simulink model "FMS"  (R2018b)
settings: configuration reference "fms_config" (kept outside this file)
values from neighbouring files (symbols this model uses):
  FMS_EXPORT = Simulink.Parameter(FMS_EXPORT_VALUE)    [fms_model_init.m]
  FMS_PARAM = Simulink.Parameter(FMS_PARAM_VALUE)    [fms_model_init.m]
undefined symbols (not defined in the file or in its folder): actuator_cmd, ax_cmd, ay_cmd, az_cmd, cmd_mask, ControlMode, ctrl_mode, DiscIntNeverNeededParam, FMS_Cmd, FMS_CONST, FMS_Error, home, mode, p_cmd, phi_cmd, PilotMode, psi_rate_cmd, q_cmd, r_cmd, reset, state, status, theta_cmd, throttle_cmd, timestamp, u_cmd, v_cmd, VehicleState, VehicleStatus, w_cmd, wp_consume, wp_current
libraries: simulink x123, FMT_Model_Lib x62, hdlsllib x13
(part 7 of 7)

== stateflow chart FMS/FMS Commander/Commander/Arm/Assist/Position/Altitude Command/Detect Movement/Motion Status ==
  state Hold
    entry:
    state=MotionState.Hold;
  state Move
    entry:
    state=MotionState.Move;
  state Brake
    entry:
    state=MotionState.Brake;
  (default) -> Move
  Hold -> Move : [motion_req==1]
  Move -> Brake : [motion_req==0]
  Brake -> Move [order 2] : [motion_req==1]
  Brake -> Hold [order 1] : [speed<=0.15 || after(1.5, sec)]
  data: state output Enum: MotionState; motion_req input; speed input

== stateflow chart FMS/FMS Commander/Commander/Arm/Auto/Mission/Mission_SubSystem/Velocity Commander/Hold Position/Altitude Hold/Detect Movement/Motion Status ==
  state Hold
    entry:
    state=MotionState.Hold;
  state Move
    entry:
    state=MotionState.Move;
  state Brake
    entry:
    state=MotionState.Brake;
  (default) -> Move
  Hold -> Move : [motion_req==1]
  Move -> Brake : [motion_req==0]
  Brake -> Move [order 2] : [motion_req==1]
  Brake -> Hold [order 1] : [speed<=0.15 || after(1.5, sec)]
  data: state output Enum: MotionState; motion_req input; speed input

== stateflow chart FMS/FMS Commander/Commander/Arm/Auto/Mission/Mission_SubSystem/Velocity Commander/Hold Position/Position Hold/Detect Movement/Motion State ==
  state Hold
    entry:
    state=MotionState.Hold;
  state Move
    entry:
    state=MotionState.Move;
  state Brake
    entry:
    state=MotionState.Brake;
  (default) -> Move
  Hold -> Move : [motion_req==1]
  Move -> Brake : [motion_req==0]
  Brake -> Move [order 2] : [motion_req==1]
  Brake -> Hold [order 1] : [speed<=0.2 || after(2.5, sec)]
  data: state output Enum: MotionState; motion_req input; speed input

== matlab function FMS/FMS Commander/Commander/Arm/Auto/Mission/Mission_SubSystem/Velocity Commander/L1 Reference WP/NearbyRefWP ==
  data: P output; P2 input; d output; P3 input; L1 input
% Find the reference waypoint when vehicle (P3) is close to target (P2)
%
% If the vehicle is close to target (distance(P2,P3) < L1), select P2 as
% reference waypoint and return the distance, otherwise return -1.
function [P,d] = NearbyRefWP(P2, P3, L1)

P3P2 = P2 - P3;
dis = sqrt(sum(P3P2.^2));

if dis <= L1
    d = dis;
    % select P2 as reference WP
    P = P2;
else
    d = single(-1);
    % unset WP
    P = single([0; 0]);
end

== stateflow chart FMS/FMS Commander/Commander/Arm/Assist/Position/Heading Command/Detect Movement/Motion State ==
  state Hold
    entry:
    state=MotionState.Hold;
  state Move
    entry:
    state=MotionState.Move;
  state Brake
    entry:
    state=MotionState.Brake;
  (default) -> Move
  Hold -> Move : [motion_req==1]
  Move -> Brake : [motion_req==0]
  Brake -> Move [order 2] : [motion_req==1]
  Brake -> Hold [order 1] : [speed<=0.1 || after(1, sec)]
  data: state output Enum: MotionState; motion_req input; speed input

== matlab function FMS/FMS Commander/Commander/Arm/Auto/Mission/Mission_SubSystem/Velocity Commander/L1 Reference WP/OutRegionRegWP ==
  data: P1 input; P output; P2 input; P3 input
% Find the reference waypoint when vehicle is out of L1 region near P1P2.
%
% There are three region defined:
%   Region 1: The project point of P3 is lied on left side of P1P2
%   Region 2: The project point of P3 is lied on right side of P1P2
%   Region 3: The project point of P3 is lied on the segment line 
%
%   For the case of region 3, we select the project point as the reference
%   wayspoint. For the case of region 1, we choose P1 as reference waypoint
%   and similarly for the case of region 2, we choose P3 as reference
%   waypoint.
function P = OutRegionRefWP(P1, P2, P3)
% segment line P1P2
P1P2 = P2 - P1;
% segment line P1P3
P1P3 = P3 - P1;

% Define C as the P3 project point on line P1P2.
% Hence, P1C = dot(P1P3, P1P2)/|P1P2| * (P1P2/|P1P2|) = u * P1P2
% where u = dot(P1P3, P1P2) / |P1P2|^2.
u = dot(P1P3, P1P2) / sum(P1P2.^2);

if u <= 0
    % region 1
    P = P1;
elseif u >= 1
    % region 2
    P = P2;
else
    % region 3. C = P1C + P1
    P = u * P1P2 + P1;
end

== matlab function FMS/FMS Commander/Commander/Arm/Auto/Mission/Mission_SubSystem/Velocity Commander/L1 Reference WP/SearchL1RefWP ==
  data: P1 input; P output; P2 input; P3 input; L1 input; u output
% Find reference waypoint (L1RefWP) on the line segment P1P2 which has 
% L1 distance from vehicle position (P3).
%
% The idea is to calculate the intersection point of a circle with L1 radius
% with the line segment P1P2.
%
% Define P = P1 + u * (P2 - P1), where P is the intersection point.
% Goal is calculating the u, where the valid u is between [0, 1].
%
% Input:
%   P1: start point of segment line
%   P2: start point of segment line
%   P3: circle center point, also is known as the vehicle position
%   L1: the L1 distance
% Output:
%   P: L1 reference waypoint
%   u: scale factor (valid between 0 and 1), -1 means no intersection.
function [P, u] = SearchL1RefWP(P1, P2, P3, L1)

% P1 = (x1, y1), P2 = (x2, y2), P3 = (x3, y3)
x1 = P1(1);
y1 = P1(2);
x2 = P2(1);
y2 = P2(2);
x3 = P3(1);
y3 = P3(2);

% The P is on circle and line segment, which yields:
A = (x2 - x1)^2 + (y2 - y1)^2;
B = 2 * ((x2 - x1)*(x1 - x3) + (y2 - y1)*(y1 - y3));
C = x3^2 + y3^2 + x1^2 + y1^2 - 2*(x3*x1 + y3*y1) - L1^2;
% Check root existence confition if B^2 - 4*A*C >= 0
D = B^2 - 4*A*C;
u = single(-1);
P = single([0 0]);

if D > 0
    % D>0 means we have 2 difference roots, % root is valid only if u is in range of [0, 1]
    u1 = (-B + sqrt(D)) / (2*A);
    u2 = (-B - sqrt(D)) / (2*A);
    
    if (u1>=0 && u1<=1) && (u2>=0 && u2<=1)
        % have 2 valid roots, select the one which is closer to P2 (target point)
        if u1 > u2
            u = u1; 
        else
            u = u2;
        end
    elseif (u1>=0 && u1<=1)
        % only 1 root valid, select it
        u = u1;
    elseif (u2>=0 && u2<=1)
        % only 1 root valid, select it
        u = u2;
    else
        % no valid root, which means no intersection point founded.
        return;
    end
elseif D == 0
    % D=0 means only 1 single root
    u1 = -B / (2*A);
    if (u1>=0 && u1<=1)
        % valid root, select it
        u = u1;
    else
        % no valid root, which means no intersection point founded.
        return;
    end
else
    % no valid root, which means no intersection point founded.
    return;
end

% calculate the L1 reference waypoint (P) coordinate
P(1) = x1 + u*(x2 - x1);
P(2) = y1 + u*(y2 - y1);

== stateflow chart FMS/FMS Commander/Commander/Arm/SubMode/Return/Velocity Commander/Hold Position/Altitude Hold/Detect Movement/Motion Status ==
  state Hold
    entry:
    state=MotionState.Hold;
  state Move
    entry:
    state=MotionState.Move;
  state Brake
    entry:
    state=MotionState.Brake;
  (default) -> Move
  Hold -> Move : [motion_req==1]
  Move -> Brake : [motion_req==0]
  Brake -> Move [order 2] : [motion_req==1]
  Brake -> Hold [order 1] : [speed<=0.15 || after(1.5, sec)]
  data: state output Enum: MotionState; motion_req input; speed input

== stateflow chart FMS/FMS State Machine ==
  state Command_Listener [parallel]
    settings: executionOrder=1
    state Send
      entry:
      % Send command
      M.data=save_cmd;
      send(M);
    state Listen
    state Check
      entry:
      valid_cmd = CheckCmdValid(save_cmd, mode, INS_Out.flag, fms_error);
    (default) -> Listen
    Send -> Listen
    Check -> Listen [order 2]
    Listen -> Check : [hasChanged(cmd) && ...
        | cmd ~= FMS_Cmd.None]{save_cmd = cmd;}
    Check -> Send [order 1] : [valid_cmd == true]
  state Vehicle [parallel]
    du:
    % if mission data updated, reset waypoint index
    if hasChanged(mission_timestamp)
    wp_consume = 0;
    wp_index = 1;
    end
    settings: executionOrder=4
    state moved = StickMoved(stick_val,pilot_cmd) [function]
    state sp_takeoff = PrepTakeoff(xy_R) [function]
    state Arm
      en:
      status = VehicleStatus.Arm;
      state SubMode
        en:
        % save enter stick value
        stick_val = [Pilot_Cmd.stick_yaw; Pilot_Cmd.stick_throttle; Pilot_Cmd.stick_roll; Pilot_Cmd.stick_pitch];
        state Return
          en:
          state = VehicleState.Return;
        state Land
          en:
          state = VehicleState.Land;
        state Takeoff
          en:
          state = VehicleState.Takeoff;
        state Hold
          en:
          state = VehicleState.Hold;
        Vehicle.Arm.SubMode.Return -> Vehicle.Arm.SubMode.Land : [norm([INS_Out.x_R,INS_Out.y_R]-[home(1),home(2)]) ...
            | <= accept_radius]
            | {Cmd_In.sp_waypoint = [home(1); home(2); 0]}
        Vehicle.Arm.SubMode.Takeoff -> (junction 612) : [INS_Out.h_R >= Cmd_In.sp_waypoint(3)]
        (junction 612) -> Vehicle.Arm.SubMode.Hold [order 2]
      state Auto
        state Offboard
          state Loiter
            en:
            state = VehicleState.Hold;
          state Run
            en:
            state = VehicleState.Offboard;
          (default) -> (junction 958)
          (junction 958) -> Vehicle.Arm.Auto.Offboard.Loiter [order 2]
          (junction 958) -> Run [order 1] : [auto_cmd_valid == 1]
          Run -> Vehicle.Arm.Auto.Offboard.Loiter : [auto_cmd_valid == 0]
          Vehicle.Arm.Auto.Offboard.Loiter -> Run : [auto_cmd_valid == 1]
        state Mission
          en:
          % Reference location of latitude and longitude, specified as an m-by-2 array, in degrees
          llo = [INS_Out.lat_0, INS_Out.lon_0] * (180/pi);
          % Set setpoint waypoint to current position
          Cmd_In.sp_waypoint = [INS_Out.x_R; INS_Out.y_R; INS_Out.h_R];
          % Init set_speed and set_yaw
          Cmd_In.set_speed = single(0);
          Cmd_In.set_yaw = single(-1);
          state pos = LLA2FLAT(lla,llo,href,psio) [function]
          state Takeoff_Waypoint
            en:
            % Geodetic coordinates (latitude, longitude, and altitude), specified as an m-by-3 array in [degrees degrees meters]
            % Altitude add home(3) here because the altitude when takeoff could be non-zero
            lla = [double(Mission_Data.x(wp_index))*1e-7, double(Mission_Data.y(wp_index))*1e-7, double(-(Mission_Data.z(wp_index) + home(3)))];
            % set takeoff setpoint
            Cmd_In.cur_waypoint = [INS_Out.x_R; INS_Out.y_R; INS_Out.h_R];
            Cmd_In.sp_waypoint = LLA2FLAT(lla, llo, 0, 0);
            % enter mission state
            state = VehicleState.Mission;
          state Loiter
            en:
            state = VehicleState.Hold;
          state NextWP
            en:
            if wp_index <= Mission_Data.valid_items
            nav_cmd = Mission_Data.command(wp_index);
            else
            nav_cmd = uint16(NAV_Cmd.None);
            % updated consumed waypoints
            wp_consume = wp_index - 1;
            end
          state Takeoff
            en:
            % Geodetic coordinates (latitude, longitude, and altitude), specified as an m-by-3 array in [degrees degrees meters]
            % Altitude add home(3) here because the altitude when takeoff could be non-zero
            lla = [double(Mission_Data.x(wp_index))*1e-7, double(Mission_Data.y(wp_index))*1e-7, double(-(Mission_Data.z(wp_index) + home(3)))];
            % set takeoff setpoint
            Cmd_In.cur_waypoint = [INS_Out.x_R; INS_Out.y_R; INS_Out.h_R];
            Cmd_In.sp_waypoint = LLA2FLAT(lla, llo, 0, 0);
            Cmd_In.sp_waypoint(1:2) = reachable_wp(Cmd_In.cur_waypoint, Cmd_In.sp_waypoint);
            % enter takeoff state
            state = VehicleState.Takeoff;
            state reachable_wp = reachable_wp(cur_waypoint,sp_waypoint) [function]
          state Waypoint
            en:
            % Geodetic coordinates (latitude, longitude, and altitude), specified as an m-by-3 array in [degrees degrees meters]
            % Altitude add home(3) here because the altitude when takeoff could be non-zero
            lla = [double(Mission_Data.x(wp_index))*1e-7, double(Mission_Data.y(wp_index))*1e-7, double(-(Mission_Data.z(wp_index) + home(3)))];
            % set current waypoint to previous setpoint waypoint
            Cmd_In.cur_waypoint = Cmd_In.sp_waypoint;
            % target waypoint
            Cmd_In.sp_waypoint = LLA2FLAT(lla, llo, 0, 0);
            % set yaw
            if Mission_Data.param4(wp_index) >= 0
            Cmd_In.set_yaw = Mission_Data.param4(wp_index)/180*pi;
            else
            Cmd_In.set_yaw = atan2(Cmd_In.sp_waypoint(2)-Cmd_In.cur_waypoint(2), Cmd_In.sp_waypoint(1)-Cmd_In.cur_waypoint(1));
            end
            state = VehicleState.Mission;
          state Disarming
          state Hold
            en:
            state = VehicleState.Hold;
          state SetSpeed
            en:
            % set cruise speed
            Cmd_In.set_speed = Mission_Data.param2(wp_index);
          state Land
            en:
            Cmd_In.sp_waypoint = [INS_Out.x_R; INS_Out.y_R; 0];
            state = VehicleState.Land;
          state Return
            en:
            Cmd_In.sp_waypoint = [home(1); home(2); INS_Out.h_R];
            state = VehicleState.Return;
          Mission -> NextWP : [hasChanged(mission_timestamp)]
          (junction 908) -> (junction 910) : {wp_index = wp_index + 1;}
          (junction 910) -> NextWP
          (junction 873) -> (junction 908)
          (default) -> NextWP
          Takeoff_Waypoint -> (junction 873) : [norm([INS_Out.x_R;INS_Out.y_R;INS_Out.h_R]-Cmd_In.sp_waypoint(1:3)) <= accept_radius]
          (junction 1010) -> Takeoff_Waypoint [order 1] : [norm([INS_Out.x_R;INS_Out.y_R]-Cmd_In.sp_waypoint(1:2)) <= accept_radius]
          NextWP -> Vehicle.Arm.Auto.Mission.Takeoff [order 1] : [nav_cmd == NAV_Cmd.Takeoff]
          Vehicle.Arm.Auto.Mission.Takeoff -> (junction 1010) : [INS_Out.h_R >= Cmd_In.sp_waypoint(3)]
          (junction 1010) -> (junction 873) [order 2]
          (junction 917) -> Vehicle.Arm.Auto.Mission.Loiter [order 2]
          (junction 879) -> (junction 873)
          NextWP -> (junction 917) [order 6]
          (junction 917) -> Disarming [order 1] : [on_ground]
          NextWP -> Waypoint [order 2] : [nav_cmd == NAV_Cmd.Waypoint]
          Waypoint -> (junction 997) : [norm([INS_Out.x_R;INS_Out.y_R;INS_Out.h_R]-Cmd_In.sp_waypoint(1:3)) <= accept_radius]
              | {Cmd_In.set_speed = single(0); Cmd_In.set_yaw = single(-1);}
          (junction 997) -> (junction 879) [order 2]
          (junction 997) -> Vehicle.Arm.Auto.Mission.Hold [order 1] : [Mission_Data.param1(wp_index) > 0]
          Vehicle.Arm.Auto.Mission.Hold -> (junction 879) : after(Mission_Data.param1(wp_index),sec)
          (junction 994) -> (junction 879)
          NextWP -> SetSpeed [order 3] : [nav_cmd == NAV_Cmd.SetSpeed]
          SetSpeed -> (junction 994)
          (junction 915) -> (junction 994)
          NextWP -> Vehicle.Arm.Auto.Mission.Return [order 5] : [nav_cmd == NAV_Cmd.Return]
          NextWP -> Vehicle.Arm.Auto.Mission.Land [order 4] : [nav_cmd == NAV_Cmd.Land]
          Vehicle.Arm.Auto.Mission.Land -> (junction 915) : [duration(on_ground) >= 2]
          Vehicle.Arm.Auto.Mission.Return -> Vehicle.Arm.Auto.Mission.Land : [norm([INS_Out.x_R; INS_Out.y_R]-Cmd_In.sp_waypoint(1:2)) < 0.5]
        state InvalidAutoMode
        (default) -> (junction 43)
        (junction 43) -> Offboard [order 1] : [mode == PilotMode.Offboard]
        (junction 43) -> (junction 134) [order 2]
        (junction 134) -> Mission [order 1] : [mode == PilotMode.Mission]
        (junction 134) -> InvalidAutoMode [order 2]
        Disarming -> (junction 370)
        InvalidAutoMode -> (junction 370)
      state Assist
        state InvalidAssistMode
        state Acro
          en:
          state = VehicleState.Acro;
        state Stabilize
          en:
          state = VehicleState.Stabilize;
        state Altitude
          en:
          state = VehicleState.Altitude;
        state Position
          en:
          state = VehicleState.Position;
        (default) -> (junction 354)
        (junction 354) -> (junction 190) [order 2]
        (junction 190) -> (junction 193) [order 2]
        (junction 193) -> (junction 196) [order 2]
        (junction 196) -> InvalidAssistMode [order 2]
        (junction 354) -> Acro [order 1] : [mode == PilotMode.Acro]
        (junction 190) -> Stabilize [order 1] : [mode == PilotMode.Stabilize]
        (junction 193) -> Altitude [order 1] : [mode == PilotMode.Altitude]
        (junction 196) -> Position [order 1] : [mode == PilotMode.Position]
      state Manual
        state InValidManualMode
        state Manual
          en:
          state = VehicleState.Manual;
        (default) -> (junction 410)
        (junction 410) -> InValidManualMode [order 2]
        (junction 410) -> Vehicle.Arm.Manual.Manual [order 1] : [mode == PilotMode.Manual]
      state InvalidArmMode
      Vehicle.Arm -> Vehicle.Arm.SubMode.Land [order 3] : M[M.data==FMS_Cmd.Land]
          | {Cmd_In.sp_waypoint = [INS_Out.x_R; INS_Out.y_R; 0]}
      Vehicle.Arm -> Vehicle.Arm.SubMode.Hold [order 1] : M[M.data==FMS_Cmd.Pause]
      Vehicle.Arm -> Vehicle.Arm.SubMode.Return [order 4] : M[M.data==FMS_Cmd.Return]
          | {Cmd_In.cur_waypoint = [INS_Out.x_R; INS_Out.y_R; INS_Out.h_R];
          | Cmd_In.sp_waypoint = [home(1); home(2); INS_Out.h_R]}
      Vehicle.Arm.SubMode.Hold -> Vehicle.Arm : M[M.data==FMS_Cmd.Continue ...
          | && mode ~= PilotMode.None]
      (junction 612) -> (junction 117) [order 1] : [mode ~= PilotMode.None]
      SubMode -> (junction 117) : [(StickMoved(stick_val, Pilot_Cmd) || ...
          | bitand(INS_Out.flag, 212) ~= 212) && ...
          | mode ~= PilotMode.None]
      Vehicle.Arm -> (junction 117) [order 2] : [hasChanged(mode) && ...
          | mode ~= PilotMode.None]
      (junction 117) -> Auto [order 1] : [getArmMode(mode) == 3]
      (default) -> (junction 117)
      (junction 117) -> (junction 140) [order 2]
      (junction 140) -> Assist [order 1] : [getArmMode(mode)  == 2]
      (junction 140) -> (junction 240) [order 2]
      (junction 240) -> Vehicle.Arm.Manual [order 1] : [getArmMode(mode)  == 1]
      (junction 240) -> InvalidArmMode [order 2]
    state Standby
      en:
      % check if mission takeoff is valid
      if mode==PilotMode.Mission
      if (wp_index <= Mission_Data.valid_items && ...
      Mission_Data.command(wp_index)==NAV_Cmd.Takeoff) || ...
      (wp_index+1 <= Mission_Data.valid_items && ...
      Mission_Data.command(wp_index)==NAV_Cmd.SetSpeed && ...
      Mission_Data.command(wp_index+1)==NAV_Cmd.Takeoff)
      % set mission takeoff flag, so enter mission mode after 2s
      prep_mission_takeoff = 1;
      % unset prep_takeoff if prep_mission_takeoff=1
      prep_takeoff = 0;
      else
      send(DisarmEvent);
      end
      end
      % set current position as home
      home = [INS_Out.x_R; INS_Out.y_R; INS_Out.h_R; INS_Out.psi];
      % enter standby state
      state = VehicleState.Standby;
      status = VehicleStatus.Standby;
      ex:
      % on exit, unset takeoff flag
      prep_takeoff = 0;
      prep_mission_takeoff = 0;
    state Disarm
      en:
      state = VehicleState.Disarm;
      status = VehicleStatus.Disarm;
    InValidManualMode -> Vehicle
    Vehicle.Arm.SubMode.Land -> (junction 330) : [duration(on_ground) >= 2]
    (junction 330) -> Vehicle.Disarm
    (junction 332) -> (junction 334)
    (junction 334) -> Vehicle.Arm.SubMode.Takeoff : {Cmd_In.cur_waypoint = [INS_Out.x_R; INS_Out.y_R; INS_Out.h_R];
        | Cmd_In.sp_waypoint = PrepTakeoff([INS_Out.x_R; INS_Out.y_R]);
        | Cmd_In.sp_waypoint(3) = Cmd_In.sp_waypoint(3) + home(3);}
    Standby -> (junction 332) [order 2] : M[M.data==FMS_Cmd.Takeoff]
    Standby -> (junction 334) [order 1] : [duration(prep_takeoff == 1) >= 2]
    (junction 989) -> Vehicle.Arm.SubMode.Hold
    (junction 987) -> (junction 989) : [pilot_cmd_lost && bitand(INS_Out.flag, 212) == 212]
    InvalidAssistMode -> Vehicle
    (junction 370) -> Vehicle
    (default) -> Vehicle.Disarm
    Assist -> (junction 987)
    Standby -> Vehicle.Disarm [order 3] : after(10, sec) || DisarmEvent
    Vehicle.Disarm -> Standby [order 1] : M[M.data==FMS_Cmd.PreArm]
    Standby -> Vehicle.Arm [order 6] : [ManualArmEvent(Pilot_Cmd) == 1 &&...
        | mode ~= PilotMode.None &&...
        | prep_takeoff ~= 1]
    Vehicle.Disarm -> Standby [order 2] : M[M.data==FMS_Cmd.Takeoff]
        | {prep_takeoff = 1;}
    Standby -> Vehicle.Arm [order 5] : [mode == PilotMode.Offboard && ...
        | auto_cmd_valid && prep_takeoff ~= 1]
    Vehicle -> Vehicle.Disarm : M[M.data==FMS_Cmd.Disarm]
    (junction 304) -> Vehicle.Disarm
    Standby -> (junction 903) [order 4] : [duration(prep_mission_takeoff == 1) >= 2]
    (junction 903) -> Vehicle.Arm
    Vehicle.Arm -> (junction 304) [order 1] : [duration(on_ground) >= 2 && mode ~= PilotMode.Mission]
    InvalidArmMode -> Vehicle
  state Combo_Stick [parallel]
    settings: executionOrder=2
    state res = BottomRight(pilot_cmd) [function]
      (default) -> (junction 285) : {res = (pilot_cmd.stick_throttle < -0.8) && ...
          | (pilot_cmd.stick_yaw > 0.8);}
    state Idle
      du:
      bl = BottomLeft(Pilot_Cmd);
      br = BottomRight(Pilot_Cmd);
    state Arm
      en:
      M.data=FMS_Cmd.PreArm;
      send(M);
    state res = BottomLeft(pilot_cmd) [function]
      (default) -> (junction 298) : {res = (pilot_cmd.stick_throttle < -0.8) && ...
          | (pilot_cmd.stick_yaw < -0.8);}
    state Disarm
      en:
      send(DisarmEvent, Vehicle)
    (default) -> Idle
    Combo_Stick.Arm -> Idle : [~BottomRight(Pilot_Cmd)]
    Idle -> Combo_Stick.Arm [order 1] : [duration(br)>1.5]
    Idle -> Combo_Stick.Disarm [order 2] : [duration(bl)>1.5]
    Combo_Stick.Disarm -> Idle : [~BottomLeft(Pilot_Cmd)]
  state Lost_Return [parallel]
    settings: executionOrder=3
    state Lost
      en:
      % check if INS valid to return
      if bitand(INS_Out.flag, 221)
      M.data=FMS_Cmd.Return;
      send(M);
      end
    state Connect
    (default) -> Connect
    Connect -> Lost : [lost_connect]
    Lost -> Connect : [~lost_connect]
  data: cmd_in function_input; mode_in function_input; valid function_output; ins_flag function_input; error function_input; pilotMode function_input; armMode function_output; pilot_cmd function_input; trigger function_output; stick_val function_input double size=4; moved function_output; pilot_cmd function_input Bus: Pilot_Cmd_Bus size=1; xy_R function_input single size=2; sp_takeoff function_output; lla function_input double size=[1 3]; llo function_input double size=[1 2]; href function_input double size=1; pos function_output; psio function_input double size=1; cur_waypoint function_input single size=3; sp_waypoint function_input single size=3; reachable_wp function_output single size=2; res function_output; pilot_cmd function_input; res function_output; pilot_cmd function_input; state output Enum: VehicleState; cmd input; valid_cmd local; M local Enum: FMS_Cmd; mode input; Pilot_Cmd input Bus: Pilot_Cmd_Bus; lost_connect input; pilot_cmd_lost input; INS_Out input Bus: INS_Out_Bus; Mission_Data input Bus: Mission_Data_Bus; prep_takeoff local =0; stick_val local; bl local =false; br local =false; nav_cmd local uint16; wp_consume output uint8 =uint8(0); wp_index output uint8 =uint8(1); Cmd_In output Bus: Commander_In_Bus; mission_timestamp input uint32 =uint32(0); on_ground input; auto_cmd_valid input; status local Enum: VehicleStatus =VehicleStatus.None; llo local; lla local; prep_mission_takeoff local =0; save_cmd local Enum: FMS_Cmd; accept_radius input; home data_store_memory; fms_error input
  events: DisarmEvent local FUNCTION_CALL_EVENT
  function valid = CheckCmdValid(cmd_in, mode_in, ins_flag, error):
    | function valid = CheckCmdValid(cmd_in, mode_in, ins_flag, error)
    | 
    | % bit1 |    bit2    |    bit3  |   bit4  | bit5  | bit6  |bit7|bit8|bit9
    | % init | standstill | attitude | heading | speed | LLA   | xy | h | h_AGL
    | 
    | valid = false;
    | 
    | % TODO: Add more checks
    | switch cmd_in
    |     case {FMS_Cmd.Takeoff, FMS_Cmd.Land, FMS_Cmd.Return, FMS_Cmd.Pause}
    |         if ~bitget(ins_flag, 1) || ~bitget(ins_flag, 3) || ~bitget(ins_flag, 4)
    |             return;
    |         end
    |         % these modes need position valid
    |         if bitget(ins_flag, 5) && bitget(ins_flag, 7) && bitget(ins_flag, 8)
    |             valid = true;
    |         end
    |         
    |         if cmd_in == FMS_Cmd.Takeoff && error ~= 0
    |            valid = false; 
    |         end
    |     case FMS_Cmd.PreArm
    |         if ~bitget(ins_flag, 1) || ~bitget(ins_flag, 3) || ~bitget(ins_flag, 4) || error ~= 0
    |             return;
    |         end
    |         
    |         switch mode_in
    |             case {PilotMode.Position, PilotMode.Mission, PilotMode.Offboard}
    |                 if bitget(ins_flag, 5) && bitget(ins_flag, 7) && bitget(ins_flag, 8)
    |                     valid = true;
    |                 end
    |             case PilotMode.Altitude
    |                 if bitget(ins_flag, 8)
    |                     valid = true;
    |                 end
    |             case PilotMode.Stabilize
    |                 valid = true;
    |             otherwise
    |                 % do nothing
    |         end
    |     case FMS_Cmd.Continue
    |         if mode_in == PilotMode.Offboard || mode_in == PilotMode.Mission
    |            valid = true; 
    |         end
    |     case FMS_Cmd.Disarm
    |         valid = true;   % always allowed disarm
    |     otherwise
    |         % do nothing
    | end
    | 
    | return;
  function armMode = getArmMode(pilotMode):
    | function armMode = getArmMode(pilotMode)
    | 
    | % Map pilot mode to arm mode
    | switch pilotMode
    |     case PilotMode.Manual
    |         armMode = 1;    % manual
    |     case {PilotMode.Acro, PilotMode.Stabilize, PilotMode.Altitude, PilotMode.Position}
    |         armMode = 2;    % asist
    |     case {PilotMode.Mission, PilotMode.Offboard}
    |         armMode = 3;    % auto
    |     otherwise
    |         armMode = 0;    % unknown
    | end
    | 
    | end
  function trigger = ManualArmEvent(pilot_cmd):
    | function trigger = ManualArmEvent(pilot_cmd)
    | 
    | trigger = 0;
    | 
    | % Map pilot mode to arm mode
    | switch pilot_cmd.mode
    |     case {PilotMode.Manual, PilotMode.Acro, PilotMode.Stabilize}
    |         if pilot_cmd.stick_throttle > -0.7
    |             trigger = 1;
    |         end
    |     case {PilotMode.Altitude, PilotMode.Position}
    |         if pilot_cmd.stick_throttle > 0.1
    |             trigger = 1;
    |         end
    |     otherwise
    |         % do nothing
    | end
    | 
    | end

== stateflow chart FMS/FMS Commander/Commander/Arm/SubMode/Hold/Altitude Hold/Detect Movement/Motion Status ==
  state Hold
    entry:
    state=MotionState.Hold;
  state Move
    entry:
    state=MotionState.Move;
  state Brake
    entry:
    state=MotionState.Brake;
  (default) -> Move
  Hold -> Move : [motion_req==1]
  Move -> Brake : [motion_req==0]
  Brake -> Move [order 2] : [motion_req==1]
  Brake -> Hold [order 1] : [speed<=0.15 || after(1.5, sec)]
  data: state output Enum: MotionState; motion_req input; speed input

== stateflow chart FMS/FMS Commander/Commander/Arm/SubMode/Hold/Heading Hold/Detect Movement/Motion State ==
  state Hold
    entry:
    state=MotionState.Hold;
  state Move
    entry:
    state=MotionState.Move;
  state Brake
    entry:
    state=MotionState.Brake;
  (default) -> Move
  Hold -> Move : [motion_req==1]
  Move -> Brake : [motion_req==0]
  Brake -> Move [order 2] : [motion_req==1]
  Brake -> Hold [order 1] : [speed<=0.1 || after(1, sec)]
  data: state output Enum: MotionState; motion_req input; speed input

== stateflow chart FMS/FMS Commander/Commander/Arm/Assist/Position/Position Command/Detect Movement/Motion State ==
  state Hold
    entry:
    state=MotionState.Hold;
  state Move
    entry:
    state=MotionState.Move;
  state Brake
    entry:
    state=MotionState.Brake;
  (default) -> Move
  Hold -> Move : [motion_req==1]
  Move -> Brake : [motion_req==0]
  Brake -> Move [order 2] : [motion_req==1]
  Brake -> Hold [order 1] : [speed<=0.25 || after(3, sec)]
  data: state output Enum: MotionState; motion_req input; speed input

== stateflow chart FMS/FMS Commander/Commander/Arm/Assist/Altitude/Altitude Command/Detect Movement/Motion Status ==
  state Hold
    entry:
    state=MotionState.Hold;
  state Move
    entry:
    state=MotionState.Move;
  state Brake
    entry:
    state=MotionState.Brake;
  (default) -> Move
  Hold -> Move : [motion_req==1]
  Move -> Brake : [motion_req==0]
  Brake -> Move [order 2] : [motion_req==1]
  Brake -> Hold [order 1] : [speed<=0.15 || after(1.5, sec)]
  data: state output Enum: MotionState; motion_req input; speed input

== stateflow chart FMS/FMS Commander/Commander/Arm/Assist/Stabilize/Heading Command/Detect Movement/Motion State ==
  state Hold
    entry:
    state=MotionState.Hold;
  state Move
    entry:
    state=MotionState.Move;
  state Brake
    entry:
    state=MotionState.Brake;
  (default) -> Move
  Hold -> Move : [motion_req==1]
  Move -> Brake : [motion_req==0]
  Brake -> Move [order 2] : [motion_req==1]
  Brake -> Hold [order 1] : [speed<=0.1 || after(1, sec)]
  data: state output Enum: MotionState; motion_req input; speed input

== stateflow chart FMS/FMS Commander/Commander/Arm/SubMode/Hold/Position Hold/Detect Movement/Motion State ==
  state Hold
    entry:
    state=MotionState.Hold;
  state Move
    entry:
    state=MotionState.Move;
  state Brake
    entry:
    state=MotionState.Brake;
  (default) -> Move
  Hold -> Move : [motion_req==1]
  Move -> Brake : [motion_req==0]
  Brake -> Move [order 2] : [motion_req==1]
  Brake -> Hold [order 1] : [speed<=0.2 || after(2.5, sec)]
  data: state output Enum: MotionState; motion_req input; speed input

== stateflow chart FMS/FMS Commander/Commander/Arm/SubMode/Return/Velocity Commander/Hold Position/Position Hold/Detect Movement/Motion State ==
  state Hold
    entry:
    state=MotionState.Hold;
  state Move
    entry:
    state=MotionState.Move;
  state Brake
    entry:
    state=MotionState.Brake;
  (default) -> Move
  Hold -> Move : [motion_req==1]
  Move -> Brake : [motion_req==0]
  Brake -> Move [order 2] : [motion_req==1]
  Brake -> Hold [order 1] : [speed<=0.2 || after(2.5, sec)]
  data: state output Enum: MotionState; motion_req input; speed input

== matlab function FMS/FMS Commander/Commander/Arm/SubMode/Return/Velocity Commander/L1 Reference WP/NearbyRefWP ==
  data: P output; P2 input; d output; P3 input; L1 input
% Find the reference waypoint when vehicle (P3) is close to target (P2)
%
% If the vehicle is close to target (distance(P2,P3) < L1), select P2 as
% reference waypoint and return the distance, otherwise return -1.
function [P,d] = NearbyRefWP(P2, P3, L1)

P3P2 = P2 - P3;
dis = sqrt(sum(P3P2.^2));

if dis <= L1
    d = dis;
    % select P2 as reference WP
    P = P2;
else
    d = single(-1);
    % unset WP
    P = single([0; 0]);
end

== matlab function FMS/FMS Commander/Commander/Arm/SubMode/Return/Velocity Commander/L1 Reference WP/OutRegionRegWP ==
  data: P1 input; P output; P2 input; P3 input
% Find the reference waypoint when vehicle is out of L1 region near P1P2.
%
% There are three region defined:
%   Region 1: The project point of P3 is lied on left side of P1P2
%   Region 2: The project point of P3 is lied on right side of P1P2
%   Region 3: The project point of P3 is lied on the segment line 
%
%   For the case of region 3, we select the project point as the reference
%   wayspoint. For the case of region 1, we choose P1 as reference waypoint
%   and similarly for the case of region 2, we choose P3 as reference
%   waypoint.
function P = OutRegionRefWP(P1, P2, P3)
% segment line P1P2
P1P2 = P2 - P1;
% segment line P1P3
P1P3 = P3 - P1;

% Define C as the P3 project point on line P1P2.
% Hence, P1C = dot(P1P3, P1P2)/|P1P2| * (P1P2/|P1P2|) = u * P1P2
% where u = dot(P1P3, P1P2) / |P1P2|^2.
u = dot(P1P3, P1P2) / sum(P1P2.^2);

if u <= 0
    % region 1
    P = P1;
elseif u >= 1
    % region 2
    P = P2;
else
    % region 3. C = P1C + P1
    P = u * P1P2 + P1;
end

== matlab function FMS/FMS Commander/Commander/Arm/SubMode/Return/Velocity Commander/L1 Reference WP/SearchL1RefWP ==
  data: P1 input; P output; P2 input; P3 input; L1 input; u output
% Find reference waypoint (L1RefWP) on the line segment P1P2 which has 
% L1 distance from vehicle position (P3).
%
% The idea is to calculate the intersection point of a circle with L1 radius
% with the line segment P1P2.
%
% Define P = P1 + u * (P2 - P1), where P is the intersection point.
% Goal is calculating the u, where the valid u is between [0, 1].
%
% Input:
%   P1: start point of segment line
%   P2: start point of segment line
%   P3: circle center point, also is known as the vehicle position
%   L1: the L1 distance
% Output:
%   P: L1 reference waypoint
%   u: scale factor (valid between 0 and 1), -1 means no intersection.
function [P, u] = SearchL1RefWP(P1, P2, P3, L1)

% P1 = (x1, y1), P2 = (x2, y2), P3 = (x3, y3)
x1 = P1(1);
y1 = P1(2);
x2 = P2(1);
y2 = P2(2);
x3 = P3(1);
y3 = P3(2);

% The P is on circle and line segment, which yields:
A = (x2 - x1)^2 + (y2 - y1)^2;
B = 2 * ((x2 - x1)*(x1 - x3) + (y2 - y1)*(y1 - y3));
C = x3^2 + y3^2 + x1^2 + y1^2 - 2*(x3*x1 + y3*y1) - L1^2;
% Check root existence confition if B^2 - 4*A*C >= 0
D = B^2 - 4*A*C;
u = single(-1);
P = single([0 0]);

if D > 0
    % D>0 means we have 2 difference roots, % root is valid only if u is in range of [0, 1]
    u1 = (-B + sqrt(D)) / (2*A);
    u2 = (-B - sqrt(D)) / (2*A);
    
    if (u1>=0 && u1<=1) && (u2>=0 && u2<=1)
        % have 2 valid roots, select the one which is closer to P2 (target point)
        if u1 > u2
            u = u1; 
        else
            u = u2;
        end
    elseif (u1>=0 && u1<=1)
        % only 1 root valid, select it
        u = u1;
    elseif (u2>=0 && u2<=1)
        % only 1 root valid, select it
        u = u2;
    else
        % no valid root, which means no intersection point founded.
        return;
    end
elseif D == 0
    % D=0 means only 1 single root
    u1 = -B / (2*A);
    if (u1>=0 && u1<=1)
        % valid root, select it
        u = u1;
    else
        % no valid root, which means no intersection point founded.
        return;
    end
else
    % no valid root, which means no intersection point founded.
    return;
end

% calculate the L1 reference waypoint (P) coordinate
P(1) = x1 + u*(x2 - x1);
P(2) = y1 + u*(y2 - y1);
